simulink model "Partie3_CBS"  (R2023b)
settings: Solver=VariableStepAuto  StartTime=0.0  StopTime=99999  RelTol=1e-3
undefined symbols (not defined in the file): graine, p1, pe, Tb
settings Model: Creator=e2404931  LastModifiedBy=e2404931
settings DataIOCC: ReturnWorkspaceOutputs=off

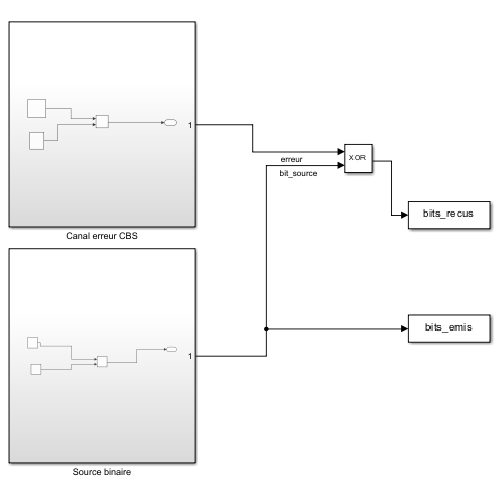
[thumbnail: Simulink's stored preview of the top-level diagram]
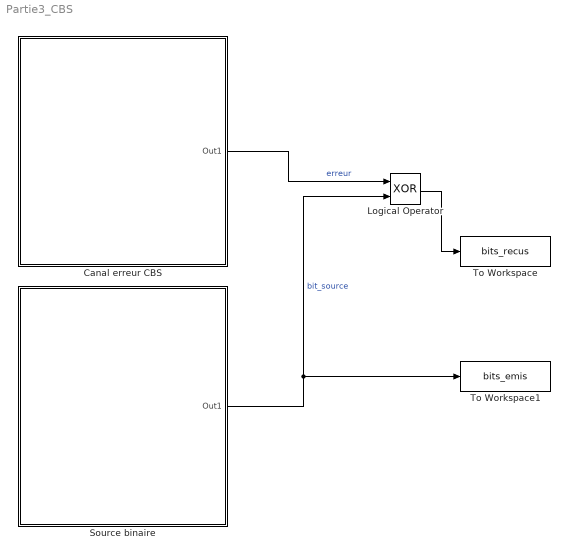
== system Partie3_CBS ==
  Canal erreur CBS : Subsystem
  Logical Operator : Logic  Operator=XOR  AllPortsSameDT=off  OutDataTypeStr=boolean
  Source binaire : Subsystem
  To Workspace : ToWorkspace  VariableName=bits_recus  SampleTime=-1
  To Workspace1 : ToWorkspace  VariableName=bits_emis  SampleTime=-1
  wires:
  Source binaire/1(Out1) -> To Workspace1/1, Logical Operator/2  "bit_source"
  Logical Operator/1 -> To Workspace/1
  Canal erreur CBS/1(Out1) -> Logical Operator/1  "erreur"

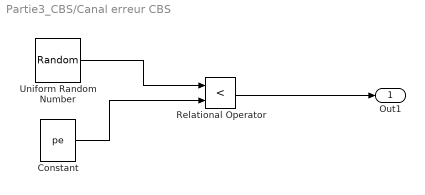
== system Partie3_CBS/Canal erreur CBS ==
  Constant : Constant  Value=pe
  Relational Operator : RelationalOperator  Operator=<  OutDataTypeStr=boolean  RndMeth=Simplest  InputSameDT=off
  Uniform Random Number : UniformRandomNumber  Minimum=0  Seed=graine+1  SampleTime=Tb
  Out1 : Outport
  wires:
  Constant/1 -> Relational Operator/2
  Uniform Random Number/1 -> Relational Operator/1
  Relational Operator/1 -> Out1/1

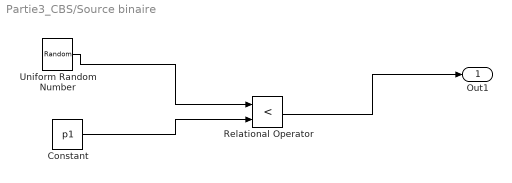
== system Partie3_CBS/Source binaire ==
  Constant : Constant  Value=p1
  Relational Operator : RelationalOperator  Operator=<  OutDataTypeStr=boolean  RndMeth=Simplest  InputSameDT=off
  Uniform Random Number : UniformRandomNumber  Minimum=0  Seed=graine  SampleTime=Tb
  Out1 : Outport
  wires:
  Uniform Random Number/1 -> Relational Operator/1
  Constant/1 -> Relational Operator/2
  Relational Operator/1 -> Out1/1
